simulink model "r2_b16a4x512f"  (R2012b)
settings: Solver=VariableStepDiscrete  SolverMode=SingleTasking  StartTime=0.0  StopTime=1  RelTol=1e-3
undefined symbols (not defined in the file): fft_stages, n_bits_ants, n_bits_xengs
libraries: xbsIndex_r4 x27410, casper_library_misc x230, xbsReplacements_r4 x24, casper_library_delays x8, xps_library x5, casper_library_communications x4
(part 69 of 229)

== system r2_b16a4x512f/sys0/vacc/bus_relational ==
  a : Inport
  b : Inport  Port=2
  a_debus : Subsystem  AncestorBlock=casper_library_flow_control/bus_expand  mask(bus_expand){mode=divisions of arbitrary size, outputNum=1, outputWidth=[1  1  1  1  1  1  1  1  1  1  1  1  1  1  1  1  1  1  1], outputBinaryPt=[0  0  0  0  0  0  0  0  0  0  0  0  0  0  0  0  0  0  0], outputArithmeticType=[0  0  0  0  0  0  0  0  0  0  0  0  0  0  0  0  0  0  0], show_format=on, outputToWorkspace=off, variablePrefix=, outputToModelAsWell=on}
      mask prompts: outputNum "Number of outputs:"; outputWidth "Output width [msb ... lsb]:"; outputBinaryPt "Output binary point position [msb ... lsb]:"; outputArithmeticType "Output arithmetic type (ufix=0, fix=1, bool=2) [msb ... lsb]:"; show_format "Print format string?"; outputToWorkspace "Output to workspace?"; variablePrefix "Variable name prefix:"; outputToModelAsWell "Output to model as well?"
      mask help:
      | Expands a 'bus' made using a bus_create or Xilinx
      | concat block.
      | The input will be divided into the specified number
      | of outputs with the specified arithmetic types.
      | Divisions are made from most significant bit.
      mask init: same as r2_b16a4x512f/bus_expand
      settings: AttributesFormatString=19 outputs: uf1.0,uf1.0,uf1.0,uf1.0,uf1.0,uf1.0,uf1.0,uf1.0,uf1.0,uf1.0,uf1.0,uf1.0,uf1.0,uf1.0,uf1.0,uf1.0,uf1.0,uf1.0,uf1.0,
      mask TypeOptions mode: divisions of equal size | divisions of arbitrary size
      mask Callback mode: bus_expand_callback();
      mask Callback outputWidth: bus_expand_callback();
      mask Callback outputToWorkspace: bus_expand_callback();
  b_debus : Subsystem  AncestorBlock=casper_library_flow_control/bus_expand  mask(bus_expand){mode=divisions of arbitrary size, outputNum=1, outputWidth=[1  1  1  1  1  1  1  1  1  1  1  1  1  1  1  1  1  1  1], outputBinaryPt=[0  0  0  0  0  0  0  0  0  0  0  0  0  0  0  0  0  0  0], outputArithmeticType=[0  0  0  0  0  0  0  0  0  0  0  0  0  0  0  0  0  0  0], show_format=on, outputToWorkspace=off, variablePrefix=, outputToModelAsWell=on}
      mask prompts: outputNum "Number of outputs:"; outputWidth "Output width [msb ... lsb]:"; outputBinaryPt "Output binary point position [msb ... lsb]:"; outputArithmeticType "Output arithmetic type (ufix=0, fix=1, bool=2) [msb ... lsb]:"; show_format "Print format string?"; outputToWorkspace "Output to workspace?"; variablePrefix "Variable name prefix:"; outputToModelAsWell "Output to model as well?"
      mask help:
      | Expands a 'bus' made using a bus_create or Xilinx
      | concat block.
      | The input will be divided into the specified number
      | of outputs with the specified arithmetic types.
      | Divisions are made from most significant bit.
      mask init: same as r2_b16a4x512f/bus_expand
      settings: AttributesFormatString=19 outputs: uf1.0,uf1.0,uf1.0,uf1.0,uf1.0,uf1.0,uf1.0,uf1.0,uf1.0,uf1.0,uf1.0,uf1.0,uf1.0,uf1.0,uf1.0,uf1.0,uf1.0,uf1.0,uf1.0,
      mask TypeOptions mode: divisions of equal size | divisions of arbitrary size
      mask Callback mode: bus_expand_callback();
      mask Callback outputWidth: bus_expand_callback();
      mask Callback outputToWorkspace: bus_expand_callback();
  bussify : Subsystem  AncestorBlock=casper_library_flow_control/bus_create  mask(bus_create){inputNum=19}
      mask prompts: inputNum "Number of inputs:"
      mask init:
      | bus_create_init(gcb,...
      |     'inputNum', inputNum);
  relational{1..19} (19 alike) : xbsIndex_r4/Relational  mode=a!=b  en=off  latency=0  dbl_ovrd=off  block_type=relational
  a!=b : Outport
  wires:
  a/1 -> a_debus/1(bus_in)
  b/1 -> b_debus/1(bus_in)
  a_debus/1(msb_out19) -> relational1/1
  b_debus/1(msb_out19) -> relational1/2
  a_debus/2(out18) -> relational2/1
  b_debus/2(out18) -> relational2/2
  a_debus/3(out17) -> relational3/1
  b_debus/3(out17) -> relational3/2
  a_debus/4(out16) -> relational4/1
  b_debus/4(out16) -> relational4/2
  a_debus/5(out15) -> relational5/1
  b_debus/5(out15) -> relational5/2
  a_debus/6(out14) -> relational6/1
  b_debus/6(out14) -> relational6/2
  a_debus/7(out13) -> relational7/1
  b_debus/7(out13) -> relational7/2
  a_debus/8(out12) -> relational8/1
  b_debus/8(out12) -> relational8/2
  a_debus/9(out11) -> relational9/1
  b_debus/9(out11) -> relational9/2
  a_debus/10(out10) -> relational10/1
  b_debus/10(out10) -> relational10/2
  a_debus/11(out9) -> relational11/1
  b_debus/11(out9) -> relational11/2
  a_debus/12(out8) -> relational12/1
  b_debus/12(out8) -> relational12/2
  a_debus/13(out7) -> relational13/1
  b_debus/13(out7) -> relational13/2
  a_debus/14(out6) -> relational14/1
  b_debus/14(out6) -> relational14/2
  a_debus/15(out5) -> relational15/1
  b_debus/15(out5) -> relational15/2
  a_debus/16(out4) -> relational16/1
  b_debus/16(out4) -> relational16/2
  a_debus/17(out3) -> relational17/1
  b_debus/17(out3) -> relational17/2
  a_debus/18(out2) -> relational18/1
  b_debus/18(out2) -> relational18/2
  a_debus/19(lsb_out1) -> relational19/1
  b_debus/19(lsb_out1) -> relational19/2
  relational1/1 -> bussify/1(in1)
  relational2/1 -> bussify/2(in2)
  relational3/1 -> bussify/3(in3)
  relational4/1 -> bussify/4(in4)
  relational5/1 -> bussify/5(in5)
  relational6/1 -> bussify/6(in6)
  relational7/1 -> bussify/7(in7)
  relational8/1 -> bussify/8(in8)
  relational9/1 -> bussify/9(in9)
  relational10/1 -> bussify/10(in10)
  relational11/1 -> bussify/11(in11)
  relational12/1 -> bussify/12(in12)
  relational13/1 -> bussify/13(in13)
  relational14/1 -> bussify/14(in14)
  relational15/1 -> bussify/15(in15)
  relational16/1 -> bussify/16(in16)
  relational17/1 -> bussify/17(in17)
  relational18/1 -> bussify/18(in18)
  relational19/1 -> bussify/19(in19)
  bussify/1(bus_out) -> a!=b/1

== system r2_b16a4x512f/sys0/vacc/flag_sampler ==
  sync : Inport
  in : Inport  Port=2
  enable : Inport  Port=3
  Constant3 : xbsIndex_r4/Constant  const=period-1  gui_display_data_type=Fixed-point  arith_type=Unsigned  n_bits=ceil(log2(period))  bin_pt=0  preci_type=Single  exp_width=8  frac_width=24  explicit_period=on  period=1  equ=P=C  opselect=C  inp2=PCIN>>17  opr=+  inp1=P  carry=CIN  dbl_ovrd=off  block_type=constant
  Counter4 : xbsIndex_r4/Counter  cnt_type=Free Running  cnt_to=Inf  operation=Up  start_count=0  cnt_by_val=1  arith_type=Unsigned  n_bits=ceil(log2(period))  bin_pt=0  load_pin=off  rst=on  en=on  explicit_period=on  period=1  dbl_ovrd=off  use_behavioral_HDL=off  implementation=Fabric  use_rpm=on  block_type=counter
      settings: xl_area=[0, 0, 0, 0, 0, 0, 0]
  Delay10 : xbsIndex_r4/Delay  rst=off  infoeditControl=Selection of Reset will increase slice count due to use of real FFs and instead of SRLs  en=off  latency=1  dbl_ovrd=off  reg_retiming=on  block_type=delay
      settings: xl_area=[0, 0, 0, 0, 0, 0, 0]
  Logical : xbsIndex_r4/Logical  logical_function=OR  inputs=2  en=off  latency=0  precision=Full  arith_type=Unsigned  n_bits=16  bin_pt=0  align_bp=on  dbl_ovrd=off  block_type=logical
  Register : xbsIndex_r4/Register  init=0  rst=off  en=on  dbl_ovrd=off  block_type=register
  Relational : xbsIndex_r4/Relational  mode=a>=b  en=off  latency=0  dbl_ovrd=off  block_type=relational
      settings: xl_area=[0, 0, 0, 0, 0, 0, 0]  block_version=10.1.3
  out : Outport
  sample_out : Outport  Port=2
  wires:
  enable/1 -> Counter4/2
  Relational/1 -> Logical/1
  Constant3/1 -> Relational/2
  Counter4/1 -> Relational/1
  Logical/1 -> Delay10/1, Counter4/1
  sync/1 -> Logical/2
  Register/1 -> out/1
  in/1 -> Register/1
  Delay10/1 -> sample_out/1, Register/2

== system r2_b16a4x512f/sys0/vacc/mcnt_sampler ==
  sync : Inport
  in : Inport  Port=2
  enable : Inport  Port=3
  Constant3 : xbsIndex_r4/Constant  const=period-1  gui_display_data_type=Fixed-point  arith_type=Unsigned  n_bits=ceil(log2(period))  bin_pt=0  preci_type=Single  exp_width=8  frac_width=24  explicit_period=on  period=1  equ=P=C  opselect=C  inp2=PCIN>>17  opr=+  inp1=P  carry=CIN  dbl_ovrd=off  block_type=constant
  Counter4 : xbsIndex_r4/Counter  cnt_type=Free Running  cnt_to=Inf  operation=Up  start_count=0  cnt_by_val=1  arith_type=Unsigned  n_bits=ceil(log2(period))  bin_pt=0  load_pin=off  rst=on  en=on  explicit_period=on  period=1  dbl_ovrd=off  use_behavioral_HDL=off  implementation=Fabric  use_rpm=on  block_type=counter
      settings: xl_area=[0, 0, 0, 0, 0, 0, 0]
  Delay10 : xbsIndex_r4/Delay  rst=off  infoeditControl=Selection of Reset will increase slice count due to use of real FFs and instead of SRLs  en=off  latency=1  dbl_ovrd=off  reg_retiming=on  block_type=delay
      settings: xl_area=[0, 0, 0, 0, 0, 0, 0]
  Logical : xbsIndex_r4/Logical  logical_function=OR  inputs=2  en=off  latency=0  precision=Full  arith_type=Unsigned  n_bits=16  bin_pt=0  align_bp=on  dbl_ovrd=off  block_type=logical
  Register : xbsIndex_r4/Register  init=0  rst=off  en=on  dbl_ovrd=off  block_type=register
  Relational : xbsIndex_r4/Relational  mode=a>=b  en=off  latency=0  dbl_ovrd=off  block_type=relational
      settings: xl_area=[0, 0, 0, 0, 0, 0, 0]  block_version=10.1.3
  out : Outport
  sample_out : Outport  Port=2
  wires:
  enable/1 -> Counter4/2
  Relational/1 -> Logical/1
  Constant3/1 -> Relational/2
  Counter4/1 -> Relational/1
  Logical/1 -> Delay10/1, Counter4/1
  sync/1 -> Logical/2
  Register/1 -> out/1
  in/1 -> Register/1
  Delay10/1 -> sample_out/1, Register/2

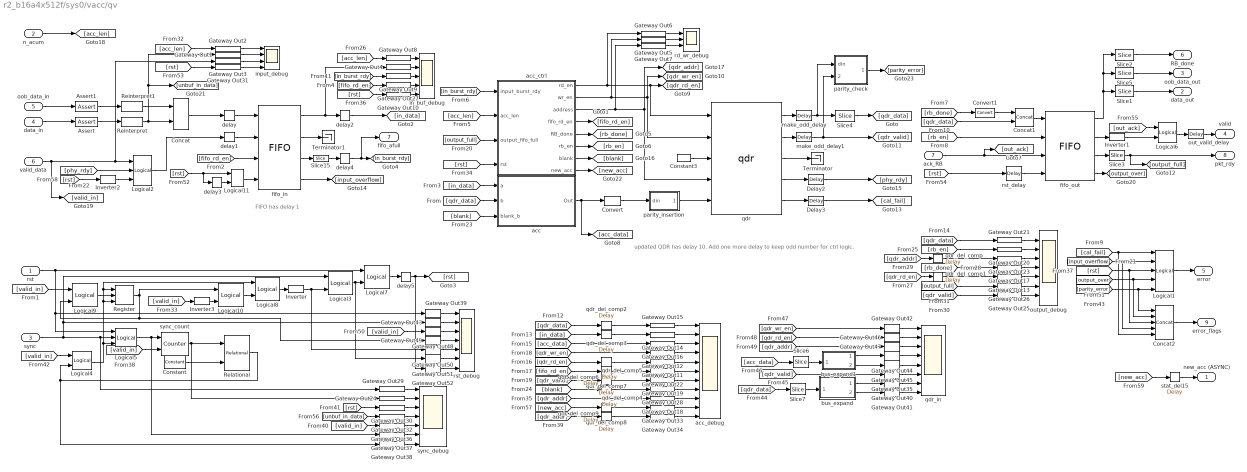
== system r2_b16a4x512f/sys0/vacc/qv ==
  note: FIFO has delay 1
  note: updated QDR has delay 10.
      | Add one more delay to keep
      | odd number for ctrl logic.
  rst : Inport
  n_acum : Inport  Port=2
  sync : Inport  Port=3
  data_in : Inport  Port=4
  oob_data_in : Inport  Port=5
  valid_data : Inport  Port=6
  ack_RB : Inport  Port=7
  Assert : xbsIndex_r4/Assert  assert_type=on  type_source=Explicitly  gui_display_data_type=Fixed-point  arith_type=Unsigned  n_bits=n_bits*2^n_inputs  bin_pt=0  preci_type=Single  exp_width=8  frac_width=24  assert_rate=off  rate_source=Explicitly  period=1  output_port=on  block_type=assert
      settings: block_version=10.1.3
  Assert1 : xbsIndex_r4/Assert  assert_type=on  type_source=Explicitly  gui_display_data_type=Fixed-point  arith_type=Unsigned  n_bits=4  bin_pt=0  preci_type=Single  exp_width=8  frac_width=24  assert_rate=on  rate_source=Explicitly  period=1  output_port=on  block_type=assert
      settings: infoedit=Asserts a user-defined sample rate and/or type on a signal.<P><P>Hardware notes: In hardware this block costs nothing.  block_version=10.1.3
  Concat : xbsIndex_r4/Concat  num_inputs=2  dbl_ovrd=off  block_type=concat
      settings: block_version=9.2.01
  Concat1 : xbsIndex_r4/Concat  num_inputs=2  dbl_ovrd=off  block_type=concat
      settings: block_version=9.2.01
  Concat2 : xbsIndex_r4/Concat  num_inputs=5  dbl_ovrd=off  block_type=concat
  Constant : xbsIndex_r4/Constant  const=vector_len-1  gui_display_data_type=Fixed-point  arith_type=Unsigned  n_bits=vector_bits  bin_pt=0  preci_type=Single  exp_width=8  frac_width=24  explicit_period=on  period=1  equ=P=C  opselect=C  inp2=PCIN>>17  opr=+  inp1=P  carry=CIN  dbl_ovrd=off  block_type=constant
  Constant3 : xbsIndex_r4/Constant  const=(2^4)-1  gui_display_data_type=Fixed-point  arith_type=Unsigned  n_bits=4  bin_pt=0  preci_type=Single  exp_width=8  frac_width=24  explicit_period=on  period=1  equ=P=C  opselect=C  inp2=PCIN>>17  opr=+  inp1=P  carry=CIN  dbl_ovrd=off  block_type=constant
      settings: block_version=9.2.01
  Convert : xbsIndex_r4/Convert  gui_display_data_type=Fixed-point  arith_type=Unsigned  n_bits=71  bin_pt=0  float_type=Single  exp_bits=8  fraction_bits=24  quantization=Truncate  overflow=Wrap  en=off  latency=0  dbl_ovrd=off  pipeline=off  block_type=convert
  Convert1 : xbsIndex_r4/Convert  gui_display_data_type=Fixed-point  arith_type=Unsigned  n_bits=1  bin_pt=0  float_type=Single  exp_bits=8  fraction_bits=24  quantization=Truncate  overflow=Wrap  en=off  latency=0  dbl_ovrd=off  pipeline=off  block_type=convert
      settings: xl_area=[0, 0, 0, 0, 0, 0, 0]  block_version=9.2.01
  Delay2 : xbsIndex_r4/Delay  rst=off  infoeditControl=Selection of Reset will increase slice count due to use of real FFs and instead of SRLs  en=off  latency=1  dbl_ovrd=off  reg_retiming=on  block_type=delay
  Delay3 : xbsIndex_r4/Delay  rst=off  infoeditControl=Selection of Reset will increase slice count due to use of real FFs and instead of SRLs  en=off  latency=1  dbl_ovrd=off  reg_retiming=on  block_type=delay
  Gateway Out{1..52} (52 alike) : xbsIndex_r4/Gateway Out  inherit_from_input=off  hdl_port=off  timing_constraint=None  locs_specified=off  LOCs={}  UseAsDAC=off  DACChannel='1'  block_type=gatewayout
      settings: infoedit="Gateway out block.  Converts Xilinx fixed point inputs into ouputs of type Simulink integer, double, or fixed point.<P><P>Hardware notes:  In hardware these blocks become top level output ports or are discarded, depending on how they are configured."  xl_area=[0, 0, 0, 0, 0, 0, 0]  block_version=10.1.3
  Inverter{,1..3} (4 alike) : xbsIndex_r4/Inverter  en=off  latency=0  dbl_ovrd=off  block_type=inv
  Logical1 : xbsIndex_r4/Logical  logical_function=OR  inputs=5  en=off  latency=1  precision=Full  arith_type=Unsigned  n_bits=16  bin_pt=0  align_bp=on  dbl_ovrd=off  block_type=logical
  Logical{3..4,6,9..10} (5 alike) : xbsIndex_r4/Logical  logical_function=AND  inputs=2  en=off  latency=0  precision=Full  arith_type=Unsigned  n_bits=16  bin_pt=0  align_bp=on  dbl_ovrd=off  block_type=logical
  Logical11 : xbsIndex_r4/Logical  logical_function=OR  inputs=2  en=off  latency=0  precision=Full  arith_type=Unsigned  n_bits=16  bin_pt=0  align_bp=on  dbl_ovrd=off  block_type=logical
  Logical2 : xbsIndex_r4/Logical  logical_function=AND  inputs=3  en=off  latency=0  precision=Full  arith_type=Unsigned  n_bits=16  bin_pt=0  align_bp=on  dbl_ovrd=off  block_type=logical
  Logical5 : xbsIndex_r4/Logical  logical_function=OR  inputs=3  en=off  latency=0  precision=Full  arith_type=Unsigned  n_bits=16  bin_pt=0  align_bp=on  dbl_ovrd=off  block_type=logical
  Logical7 : xbsIndex_r4/Logical  logical_function=OR  inputs=2  en=off  latency=0  precision=Full  arith_type=Unsigned  n_bits=16  bin_pt=0  align_bp=on  dbl_ovrd=off  block_type=logical
  Logical8 : xbsIndex_r4/Logical  logical_function=OR  inputs=2  en=off  latency=0  precision=Full  arith_type=Unsigned  n_bits=16  bin_pt=0  align_bp=on  dbl_ovrd=off  block_type=logical
  Register : xbsIndex_r4/Register  init=0  rst=on  en=on  dbl_ovrd=off  block_type=register
      settings: block_version=11.4
  Reinterpret : xbsIndex_r4/Reinterpret  force_arith_type=on  arith_type=Unsigned  force_bin_pt=on  bin_pt=0  block_type=reinterpret
      settings: block_version=9.2.01
  Reinterpret1 : xbsIndex_r4/Reinterpret  force_arith_type=on  arith_type=Unsigned  force_bin_pt=on  bin_pt=0  block_type=reinterpret
      settings: infoedit="Changes signal type without altering the binary representation.   You can changed the signal between signed and unsigned, and relocate the binary point.<P><P>Hardware notes: In hardware this block costs nothing.<P><P>Example:  Suppose the input is 6 bits wide, signed, with 2 fractional bits, and the output is forced to unsigned with 0 fractional bits.  Then an input of -2.0 (1110.00 in binary 2's complement) becomes an output of 56 (111000 in binary)."  block_version=9.2.01
  Relational : xbsIndex_r4/Relational  mode=a>=b  en=off  latency=0  dbl_ovrd=off  block_type=relational
      settings: block_version=10.1.3
  Slice1 : xbsIndex_r4/Slice  nbits=n_bits*2^n_inputs  boolean_output=off  mode=Lower Bit Location + Width  bit1=96  base1=MSB of Input  bit0=0  base0=LSB of Input  dbl_ovrd=off  block_type=slice
      settings: block_version=9.2.01
  Slice15 : xbsIndex_r4/Slice  nbits=1  boolean_output=on  mode=Upper Bit Location + Width  bit1=0  base1=MSB of Input  bit0=0  base0=LSB of Input  dbl_ovrd=off  block_type=slice
      settings: infoedit="Extracts a given range of bits from each input sample and presents it at the output.  The output type is ordinarily unsigned with binary point at zero, but can be Boolean when the slice is one bit wide.<P><P>Hardware notes: In hardware this block costs nothing."  block_version=9.2.01
  Slice2 : xbsIndex_r4/Slice  nbits=1  boolean_output=on  mode=Lower Bit Location + Width  bit1=-1  base1=MSB of Input  bit0=(2^n_inputs*n_bits)+4  base0=LSB of Input  dbl_ovrd=off  block_type=slice
      settings: block_version=9.2.01
  Slice3 : xbsIndex_r4/Slice  nbits=1  boolean_output=on  mode=Upper Bit Location + Width  bit1=0  base1=MSB of Input  bit0=0  base0=LSB of Input  dbl_ovrd=off  block_type=slice
      settings: infoedit="Extracts a given range of bits from each input sample and presents it at the output.  The output type is ordinarily unsigned with binary point at zero, but can be Boolean when the slice is one bit wide.<P><P>Hardware notes: In hardware this block costs nothing."  block_version=9.2.01
  Slice4 : xbsIndex_r4/Slice  nbits=(n_bits*2^n_inputs)+4  boolean_output=off  mode=Lower Bit Location + Width  bit1=96  base1=MSB of Input  bit0=0  base0=LSB of Input  dbl_ovrd=off  block_type=slice
      settings: block_version=9.2.01
  Slice5 : xbsIndex_r4/Slice  nbits=4  boolean_output=off  mode=Lower Bit Location + Width  bit1=96  base1=MSB of Input  bit0=n_bits*n_inputs  base0=LSB of Input  dbl_ovrd=off  block_type=slice
      settings: block_version=9.2.01
  Slice6 : xbsIndex_r4/Slice  nbits=(n_bits*2^n_inputs)  boolean_output=off  mode=Lower Bit Location + Width  bit1=96  base1=MSB of Input  bit0=0  base0=LSB of Input  dbl_ovrd=off  block_type=slice
      settings: block_version=9.2.01
  Slice7 : xbsIndex_r4/Slice  nbits=(n_bits*2^n_inputs)  boolean_output=off  mode=Lower Bit Location + Width  bit1=96  base1=MSB of Input  bit0=0  base0=LSB of Input  dbl_ovrd=off  block_type=slice
      settings: block_version=9.2.01
  Terminator : Terminator
  Terminator1 : Terminator
  acc : Subsystem  mask{n_inputs=2^n_inputs, n_bits=n_bits}
      mask prompts: n_inputs "Simultaneous inputs"; n_bits "Data width"
  acc_ctrl : Subsystem  mask{delay_qdr=11, delay_in_fifo=1, delay_adder=2}
      mask prompts: delay_qdr "delay qdr"
      mask help: QDR delay must be odd (9 is ok, 11 is ok, 10 is not).
  acc_debug : Scope  NumInputPorts=11
      settings: TimeRange=57000  YMin=0~0~0~0~0~0~0~1~1540~-1~1540  YMax=7.5e+15~7.5e+15~7.5e+15~1~1~1~1~1~1555~1~1555  SaveName=ScopeData4
  bus_expand : Subsystem  AncestorBlock=casper_library_flow_control/bus_expand  mask(bus_expand){mode=divisions of arbitrary size, outputNum=1, outputWidth=[32 32], outputBinaryPt=[14 14], outputArithmeticType=[1 1], show_format=off, outputToWorkspace=off, variablePrefix=out, outputToModelAsWell=on}
      mask prompts: outputNum "Number of outputs:"; outputWidth "Output width [msb ... lsb]:"; outputBinaryPt "Output binary point position [msb ... lsb]:"; outputArithmeticType "Output arithmetic type (ufix=0, fix=1, bool=2) [msb ... lsb]:"; show_format "Print format string?"; outputToWorkspace "Output to workspace?"; variablePrefix "Variable name prefix:"; outputToModelAsWell "Output to model as well?"
      mask help:
      | Expands a 'bus' made using a bus_create or Xilinx
      | concat block.
      | The input will be divided into the specified number
      | of outputs with the specified arithmetic types.
      | Divisions are made from most significant bit.
      mask init: same as r2_b16a4x512f/bus_expand
      settings: AttributesFormatString=2 outputs
      mask TypeOptions mode: divisions of equal size | divisions of arbitrary size
      mask Callback mode: bus_expand_callback();
      mask Callback outputWidth: bus_expand_callback();
      mask Callback outputToWorkspace: bus_expand_callback();
  bus_expand1 : Subsystem  AncestorBlock=casper_library_flow_control/bus_expand  mask(bus_expand){mode=divisions of arbitrary size, outputNum=1, outputWidth=[32 32], outputBinaryPt=[14 14], outputArithmeticType=[1 1], show_format=off, outputToWorkspace=off, variablePrefix=out, outputToModelAsWell=on}
      mask prompts: outputNum "Number of outputs:"; outputWidth "Output width [msb ... lsb]:"; outputBinaryPt "Output binary point position [msb ... lsb]:"; outputArithmeticType "Output arithmetic type (ufix=0, fix=1, bool=2) [msb ... lsb]:"; show_format "Print format string?"; outputToWorkspace "Output to workspace?"; variablePrefix "Variable name prefix:"; outputToModelAsWell "Output to model as well?"
      mask help:
      | Expands a 'bus' made using a bus_create or Xilinx
      | concat block.
      | The input will be divided into the specified number
      | of outputs with the specified arithmetic types.
      | Divisions are made from most significant bit.
      mask init: same as r2_b16a4x512f/bus_expand
      settings: AttributesFormatString=2 outputs
      mask TypeOptions mode: divisions of equal size | divisions of arbitrary size
      mask Callback mode: bus_expand_callback();
      mask Callback outputWidth: bus_expand_callback();
      mask Callback outputToWorkspace: bus_expand_callback();
  delay{,1..5} (6 alike) : xbsIndex_r4/Delay  rst=off  infoeditControl=Selection of Reset will increase slice count due to use of real FFs and instead of SRLs  en=off  latency=1  dbl_ovrd=off  reg_retiming=on  block_type=delay
  fifo_in : xbsIndex_r4/FIFO  mem_type=Distributed RAM  performance_options=Standard_FIFO  infoedit1=Available only for V4, V5, V6, V7, K7, A7 and Zynq devices.  embedded_registers=off  depth=64  percent_nbits=1  rst=on  en=off  use_dcount=off  use_percent_full_port=on  use_almost_empty=off  almost_empty_thresh=2  use_almost_full=off  almost_full_thresh=14  dbl_ovrd=off  explicit_period=off  block_type=fifo
      settings: block_version=10.1.3
  fifo_out : xbsIndex_r4/FIFO  mem_type=Block RAM  performance_options=Standard_FIFO  infoedit1=Available only for V4, V5, V6, V7, K7, A7 and Zynq devices.  embedded_registers=off  depth=1K  percent_nbits=1  rst=on  en=off  use_dcount=off  use_percent_full_port=on  use_almost_empty=off  almost_empty_thresh=2  use_almost_full=off  almost_full_thresh=14  dbl_ovrd=off  explicit_period=off  block_type=fifo
      settings: block_version=10.1.3
  in_buf_debug : Scope  NumInputPorts=5
      settings: YMin=7.6~-1~-1~-1~-1  YMax=8.4~1~1~1~1  SaveName=ScopeData2
  input_debug : Scope  NumInputPorts=4
      settings: YMin=12000~0~-5~-5  YMax=13300~1~5~5
  make_odd_delay : xbsIndex_r4/Delay  rst=off  infoeditControl=Selection of Reset will increase slice count due to use of real FFs and instead of SRLs  en=off  latency=1  dbl_ovrd=off  reg_retiming=on  block_type=delay
  make_odd_delay1 : xbsIndex_r4/Delay  rst=off  infoeditControl=Selection of Reset will increase slice count due to use of real FFs and instead of SRLs  en=off  latency=1  dbl_ovrd=off  reg_retiming=on  block_type=delay
  out_valid_delay : xbsIndex_r4/Delay  rst=off  infoeditControl=Selection of Reset will increase slice count due to use of real FFs and instead of SRLs  en=off  latency=1  dbl_ovrd=off  reg_retiming=on  block_type=delay
  output_debug : Scope  NumInputPorts=7
      settings: YMin=0~0~0~-1~0~-1~0.95  YMax=2.5e+16~1~9000~1~1~1~1.05  SaveName=ScopeData3
  parity_check : Subsystem
  parity_insertion : Subsystem
  qdr : xps_library/qdr  Tag=xps:qdr  which_qdr=qdr0  qdr_awidth=vector_bits  use_sniffer=on
      link override convert_be: n_bits=8
      link override convert_data_in: n_bits=72
      link override convert_data_in1: n_bits=72
      link override extract_parity: bitexpr=b = {a[71:0]}  arith_type1=Unsigned  arith_type2=Unsigned  arith_type3=Unsigned  arith_type4=Unsigned
      link override insert_parity: bitexpr=b = {a[71:0]}  arith_type1=Unsigned  arith_type2=Unsigned  arith_type3=Unsigned  arith_type4=Unsigned
      link override qdr_sim_model/Dual Port RAM: depth=2^qdr_awidth  initVector=[1:2^qdr_awidth]  distributed_mem=Block RAM  init_a=0  init_b=0  rst_a=off  rst_b=off  en_a=off  en_b=off  latency=1  write_mode_A=Read Before Write  write_mode_B=Read Before Write  dbl_ovrd=off  optimize=Area
      link override qdr_sim_model/sim_data_in: n_bits=72
      link override r2_2f_4x_4a_4k_r366_vacc0_qv_qdr_data_out: n_bits=72
      link override r2_4a4x128f_sys0_vacc_qv_qdr_data_out: n_bits=72
      link override r2_4a4x2kf_sys0_vacc_qv_qdr_data_out: n_bits=72
      link override r2_b4a4x256f_4gbe_sys0_vacc_qv_qdr_data_out: n_bits=72
      link override r2_b4a4x256f_sys0_vacc_qv_qdr_data_out: n_bits=72
      link override x_nd_full_sys0_vacc0_qv_qdr_data_out: n_bits=72
      link override x_nd_full_sys2_vacc0_qv_qdr_data_out: n_bits=72
      link override x_nd_inc_sys2_vacc0_qv_qdr_data_out: n_bits=72
      link override x_new_bc_sys0_vacc0_qv_qdr_data_out: n_bits=72
      link override xeng_sim_vacc0_qv_qdr_data_out: n_bits=72
  qdr_del_comp : xbsIndex_r4/Delay  rst=off  infoeditControl=Selection of Reset will increase slice count due to use of real FFs and instead of SRLs  en=off  latency=11  dbl_ovrd=off  reg_retiming=on  block_type=delay
  qdr_del_comp1 : xbsIndex_r4/Delay  rst=off  infoeditControl=Selection of Reset will increase slice count due to use of real FFs and instead of SRLs  en=off  latency=11  dbl_ovrd=off  reg_retiming=on  block_type=delay
  qdr_del_comp{2..4,6} (4 alike) : xbsIndex_r4/Delay  rst=off  infoeditControl=Selection of Reset will increase slice count due to use of real FFs and instead of SRLs  en=off  latency=2  dbl_ovrd=off  reg_retiming=on  block_type=delay
  qdr_del_comp5 : xbsIndex_r4/Delay  rst=off  infoeditControl=Selection of Reset will increase slice count due to use of real FFs and instead of SRLs  en=off  latency=13  dbl_ovrd=off  reg_retiming=on  block_type=delay
  qdr_del_comp7 : xbsIndex_r4/Delay  rst=off  infoeditControl=Selection of Reset will increase slice count due to use of real FFs and instead of SRLs  en=off  latency=3  dbl_ovrd=off  reg_retiming=on  block_type=delay
  qdr_del_comp8 : xbsIndex_r4/Delay  rst=off  infoeditControl=Selection of Reset will increase slice count due to use of real FFs and instead of SRLs  en=off  latency=13  dbl_ovrd=off  reg_retiming=on  block_type=delay
  qdr_del_comp9 : xbsIndex_r4/Delay  rst=off  infoeditControl=Selection of Reset will increase slice count due to use of real FFs and instead of SRLs  en=off  latency=13  dbl_ovrd=off  reg_retiming=on  block_type=delay
  qdr_in : Scope  NumInputPorts=8
      settings: TimeRange=57000  YMin=0~0~2407.5~0~-1~0~0~0  YMax=1~1~2422.5~100~1~1~200~0.0075  SaveName=ScopeData14
  rd_wr_debug : Scope  NumInputPorts=3
      settings: YMin=0~0~0  YMax=1~1~1050
  rst_debug : Scope  NumInputPorts=7
      settings: YMin=7.6~-1~-1~-1~-1~-5~-5  YMax=8.4~1~1~1~1~5~5  SaveName=ScopeData16
  rst_delay : xbsIndex_r4/Delay  rst=off  infoeditControl=Selection of Reset will increase slice count due to use of real FFs and instead of SRLs  en=off  latency=1  dbl_ovrd=off  reg_retiming=on  block_type=delay
  stat_del15 : xbsIndex_r4/Delay  rst=off  infoeditControl=Selection of Reset will increase slice count due to use of real FFs and instead of SRLs  en=off  latency=1  dbl_ovrd=off  reg_retiming=on  block_type=delay
  sync_count : xbsIndex_r4/Counter  cnt_type=Free Running  cnt_to=Inf  operation=Up  start_count=0  cnt_by_val=1  arith_type=Unsigned  n_bits=vector_bits  bin_pt=0  load_pin=off  rst=on  en=on  explicit_period=on  period=1  dbl_ovrd=off  use_behavioral_HDL=on  implementation=Fabric  use_rpm=on  block_type=counter
  sync_debug : Scope  NumInputPorts=7
      settings: YMin=-1~1090~-1~-1~0~-1~-1  YMax=1~1090~1~1~1~1~1  SaveName=ScopeData7
  new_acc (ASYNC) : Outport
  data_out : Outport  Port=2
  oob_data_out : Outport  Port=3
  valid : Outport  Port=4
  error : Outport  Port=5
  RB_done : Outport  Port=6
  fifo_afull : Outport  Port=7
  pkt_rdy : Outport  Port=8
  error_flags : Outport  Port=9
  wires:
  delay5/1 -> Gateway Out52/1, [rst]
  delay4/1 -> [in_burst_rdy], fifo_afull/1
  delay2/1 -> [in_data]
  qdr_del_comp9/1 -> Gateway Out34/1
  Gateway Out34/1 -> acc_debug/11
  [qdr_addr] -> qdr_del_comp9/1
  qdr_del_comp1/1 -> Gateway Out13/1
  qdr_del_comp/1 -> Gateway Out23/1
  make_odd_delay1/1 -> [qdr_valid], parity_check/2(valid)
  make_odd_delay/1 -> parity_check/1(din), Slice4/1
  Reinterpret1/1 -> Concat/1
  Reinterpret/1 -> Gateway Out1/1, [unbuf_in_data], Concat/2
  Assert1/1 -> Reinterpret1/1
  Assert/1 -> Reinterpret/1
  [in_data] -> acc/1(a)
  [rst] -> Gateway Out10/1
  Gateway Out10/1 -> in_buf_debug/5
  Gateway Out18/1 -> acc_debug/9
  [qdr_addr] -> Gateway Out18/1
  [rst] -> acc_ctrl/4(rst)
  [acc_len] -> Gateway Out2/1
  [acc_len] -> Gateway Out8/1
  [acc_len] -> acc_ctrl/2(acc_len)
  oob_data_in/1 -> Assert1/1
  n_acum/1 -> [acc_len]
  Gateway Out23/1 -> output_debug/3
  [qdr_addr] -> qdr_del_comp/1
  Gateway Out26/1 -> output_debug/6
  [rb_done] -> Gateway Out17/1
  [rb_en] -> Gateway Out20/1
  Gateway Out25/1 -> output_debug/7
  Gateway Out13/1 -> output_debug/5
  Gateway Out17/1 -> output_debug/4
  Gateway Out20/1 -> output_debug/2
  Gateway Out21/1 -> output_debug/1
  [output_full] -> Gateway Out26/1
  [qdr_valid] -> Gateway Out25/1
  [qdr_rd_en] -> qdr_del_comp1/1
  [qdr_data] -> Gateway Out21/1
  Gateway Out28/1 -> acc_debug/8
  Gateway Out19/1 -> acc_debug/7
  Gateway Out22/1 -> acc_debug/6
  Gateway Out11/1 -> acc_debug/5
  Gateway Out12/1 -> acc_debug/4
  Gateway Out16/1 -> acc_debug/3
  Gateway Out14/1 -> acc_debug/2
  Gateway Out15/1 -> acc_debug/1
  [blank] -> qdr_del_comp4/1
  [blank] -> acc/3(blank_b)
  acc_ctrl/7(blank) -> [blank]
  [qdr_data] -> acc/2(b)
  fifo_out/4 -> [output_over]
  qdr/3 -> Terminator/1
  [phy_rdy] -> Logical2/2
  Logical2/1 -> delay1/1
  Delay3/1 -> [cal_fail]
  Delay2/1 -> [phy_rdy]
  qdr/4 -> Delay2/1
  fifo_in/4 -> [input_overflow]
  qdr/5 -> Delay3/1
  Logical1/1 -> error/1
  acc_ctrl/5(RB_done) -> [rb_done]
  acc_ctrl/6(rb_en) -> [rb_en]
  fifo_out/3 -> Slice3/1
  [output_full] -> acc_ctrl/3(output_fifo_full)
  [qdr_valid] -> qdr_del_comp6/1
  qdr/2 -> make_odd_delay1/1
  [qdr_wr_en] -> Gateway Out12/1
  [fifo_rd_en] -> qdr_del_comp7/1
  [qdr_rd_en] -> qdr_del_comp5/1
  [acc_data] -> Gateway Out16/1
  [in_data] -> qdr_del_comp3/1
  [qdr_data] -> qdr_del_comp2/1
  Slice5/1 -> oob_data_out/1
  [in_burst_rdy] -> Gateway Out9/1
  [fifo_rd_en] -> Gateway Out27/1
  Gateway Out27/1 -> in_buf_debug/4
  Gateway Out9/1 -> in_buf_debug/3
  Gateway Out4/1 -> in_buf_debug/2
  Gateway Out8/1 -> in_buf_debug/1
  Gateway Out3/1 -> input_debug/3
  Gateway Out1/1 -> input_debug/2
  Gateway Out2/1 -> input_debug/1
  acc/1(Out) -> Convert/1, [acc_data]
  Gateway Out7/1 -> rd_wr_debug/3
  Gateway Out5/1 -> rd_wr_debug/2
  Gateway Out6/1 -> rd_wr_debug/1
  Slice2/1 -> RB_done/1
  fifo_out/1 -> Slice5/1, Slice2/1, Slice1/1
  Convert1/1 -> Concat1/1
  [rb_done] -> Convert1/1
  Concat1/1 -> fifo_out/1
  [qdr_data] -> Concat1/2
  [rb_en] -> fifo_out/2
  ack_RB/1 -> [out_ack], fifo_out/3
  [out_ack] -> Logical6/1
  Slice15/1 -> delay4/1
  [in_burst_rdy] -> acc_ctrl/1(input_burst_rdy)
  fifo_in/1 -> Gateway Out4/1, delay2/1
  acc_ctrl/4(fifo_rd_en) -> [fifo_rd_en]
  Constant3/1 -> qdr/3
  qdr/1 -> make_odd_delay/1
  acc_ctrl/3(address) -> Gateway Out7/1, qdr/4, [qdr_addr]
  acc_ctrl/2(wr_en) -> Gateway Out5/1, qdr/2, [qdr_wr_en]
  acc_ctrl/1(rd_en) -> Gateway Out6/1, qdr/1, [qdr_rd_en]
  Concat/1 -> delay/1
  valid_data/1 -> Logical2/1, Gateway Out3/1, [valid_in]
  data_in/1 -> Assert/1
  fifo_in/3 -> Slice15/1
  [cal_fail] -> Concat2/5, Logical1/1
  [input_overflow] -> Concat2/4, Logical1/2
  [rst] -> Concat2/3, Logical1/3
  [output_over] -> Logical1/4, Concat2/2
  Slice1/1 -> data_out/1
  Gateway Out31/1 -> input_debug/4
  [rst] -> Gateway Out31/1
  [rst] -> rst_delay/1
  Inverter1/1 -> Logical6/2
  fifo_out/2 -> Inverter1/1
  Logical6/1 -> out_valid_delay/1
  qdr_del_comp2/1 -> Gateway Out15/1
  qdr_del_comp3/1 -> Gateway Out14/1
  qdr_del_comp4/1 -> Gateway Out28/1
  qdr_del_comp5/1 -> Gateway Out11/1
  qdr_del_comp6/1 -> Gateway Out19/1
  qdr_del_comp7/1 -> Gateway Out22/1
  [fifo_rd_en] -> fifo_in/3
  rst_delay/1 -> fifo_out/4
  fifo_in/2 -> Terminator1/1
  delay/1 -> fifo_in/1
  delay1/1 -> fifo_in/2
  acc_ctrl/8(new_acc) -> [new_acc]
  [new_acc] -> stat_del15/1
  stat_del15/1 -> new_acc (ASYNC)/1
  [new_acc] -> qdr_del_comp8/1
  Gateway Out33/1 -> acc_debug/10
  qdr_del_comp8/1 -> Gateway Out33/1
  out_valid_delay/1 -> valid/1
  Inverter2/1 -> Logical2/3
  [rst] -> Inverter2/1
  Slice3/1 -> [output_full], pkt_rdy/1
  Constant/1 -> Relational/2
  Relational/1 -> Logical4/2, Gateway Out38/1
  sync_count/1 -> Gateway Out24/1, Relational/1
  Gateway Out30/1 -> sync_debug/3
  Gateway Out24/1 -> sync_debug/2
  Gateway Out29/1 -> sync_debug/1
  [valid_in] -> sync_count/2
  Gateway Out32/1 -> sync_debug/4
  [unbuf_in_data] -> Gateway Out32/1
  Logical7/1 -> delay5/1
  Gateway Out36/1 -> sync_debug/5
  [valid_in] -> Gateway Out36/1
  Gateway Out37/1 -> sync_debug/6
  Gateway Out38/1 -> sync_debug/7
  sync/1 -> Logical5/2, Gateway Out29/1, Gateway Out43/1, Logical3/1
  [valid_in] -> Logical4/1
  Logical5/1 -> sync_count/1, Gateway Out37/1
  Inverter/1 -> Gateway Out50/1, Logical3/2
  Logical4/1 -> Register/3, Logical8/1, Register/1, Logical5/3
  Logical3/1 -> Gateway Out51/1, Logical7/2
  [rst] -> Gateway Out30/1
  rst/1 -> Logical7/1, Gateway Out39/1, Logical5/1
  Logical8/1 -> Inverter/1
  Register/1 -> Gateway Out49/1, Logical9/2, Logical10/1
  [valid_in] -> Logical9/1
  Logical9/1 -> Register/2
  Inverter3/1 -> Logical10/2
  Logical10/1 -> Logical8/2
  [valid_in] -> Inverter3/1
  delay3/1 -> Logical11/2
  Logical11/1 -> fifo_in/4
  [rst] -> delay3/1, Logical11/1
  Convert/1 -> parity_insertion/1(din)
  parity_insertion/1(dout) -> qdr/5
  [parity_error] -> Concat2/1, Logical1/5
  Slice4/1 -> [qdr_data]
  [qdr_valid] -> Gateway Out35/1
  [qdr_data] -> Slice7/1
  bus_expand/2(lsb_out1) -> Gateway Out41/1
  [qdr_wr_en] -> Gateway Out42/1
  [acc_data] -> Slice6/1
  bus_expand1/2(lsb_out1) -> Gateway Out45/1
  bus_expand1/1(msb_out2) -> Gateway Out44/1
  [qdr_rd_en] -> Gateway Out46/1
  [qdr_addr] -> Gateway Out47/1
  Slice6/1 -> bus_expand1/1(bus_in)
  Slice7/1 -> bus_expand/1(bus_in)
  bus_expand/1(msb_out2) -> Gateway Out40/1
  Gateway Out45/1 -> qdr_in/5
  Gateway Out47/1 -> qdr_in/3
  Gateway Out42/1 -> qdr_in/1
  Gateway Out35/1 -> qdr_in/6
  Gateway Out44/1 -> qdr_in/4
  Gateway Out46/1 -> qdr_in/2
  Gateway Out40/1 -> qdr_in/7
  Gateway Out41/1 -> qdr_in/8
  Gateway Out39/1 -> rst_debug/1
  Gateway Out43/1 -> rst_debug/2
  [valid_in] -> Gateway Out48/1
  Gateway Out48/1 -> rst_debug/3
  Gateway Out49/1 -> rst_debug/4
  Gateway Out50/1 -> rst_debug/5
  Gateway Out51/1 -> rst_debug/6
  Gateway Out52/1 -> rst_debug/7
  parity_check/1(error) -> [parity_error]
  Concat2/1 -> error_flags/1

== system r2_b16a4x512f/sys0/vacc/rst_replicate ==
  in : Inport
  bussify : Subsystem  AncestorBlock=casper_library_flow_control/bus_create  mask(bus_create){inputNum=19}
      mask prompts: inputNum "Number of inputs:"
      mask init:
      | bus_create_init(gcb,...
      |     'inputNum', inputNum);
  out : Outport
  wires:
  in/1 -> bussify/1(in1), bussify/2(in2), bussify/3(in3), bussify/4(in4), bussify/5(in5), bussify/6(in6), bussify/7(in7), bussify/8(in8), bussify/9(in9), bussify/10(in10), bussify/11(in11), bussify/12(in12), bussify/13(in13), bussify/14(in14), bussify/15(in15), bussify/16(in16), bussify/17(in17), bussify/18(in18), bussify/19(in19)
  bussify/1(bus_out) -> out/1

== system r2_b16a4x512f/sys0/vacc/vacc_rst ==
  rst : Inport
  arm : Inport  Port=2
  load_time : Inport  Port=3
  current_time : Inport  Port=4
  immediate : Inport  Port=5
  Delay : xbsIndex_r4/Delay  rst=off  infoeditControl=Selection of Reset will increase slice count due to use of real FFs and instead of SRLs  en=off  latency=1  dbl_ovrd=off  reg_retiming=on  block_type=delay
  Gateway Out{,1..3} (4 alike) : xbsIndex_r4/Gateway Out  inherit_from_input=off  hdl_port=on  timing_constraint=None  locs_specified=off  LOCs={}  UseAsDAC=off  DACChannel='1'  block_type=gatewayout
  Logical : xbsIndex_r4/Logical  logical_function=OR  inputs=2  en=off  latency=0  precision=Full  arith_type=Unsigned  n_bits=16  bin_pt=0  align_bp=on  dbl_ovrd=off  block_type=logical
  Logical1 : xbsIndex_r4/Logical  logical_function=AND  inputs=2  en=off  latency=0  precision=Full  arith_type=Unsigned  n_bits=16  bin_pt=0  align_bp=on  dbl_ovrd=off  block_type=logical
  Logical2 : xbsIndex_r4/Logical  logical_function=OR  inputs=2  en=off  latency=0  precision=Full  arith_type=Unsigned  n_bits=16  bin_pt=0  align_bp=on  dbl_ovrd=off  block_type=logical
  Register2 : xbsIndex_r4/Register  init=0  rst=off  en=on  dbl_ovrd=off  block_type=register
  Register3 : xbsIndex_r4/Register  init=0  rst=on  en=on  dbl_ovrd=off  block_type=register
  Relational : xbsIndex_r4/Relational  mode=a=b  en=off  latency=1  dbl_ovrd=off  block_type=relational
      settings: block_version=10.1.3
  Scope : Scope  NumInputPorts=4
      settings: YMin=-5~-5~-5~-5  YMax=5~5~5~5  SaveName=ScopeData11
  armed : xbsIndex_r4/Register  init=0  rst=on  en=on  dbl_ovrd=off  block_type=register
  count0 : xbsIndex_r4/Counter  cnt_type=Free Running  cnt_to=Inf  operation=Up  start_count=0  cnt_by_val=1  arith_type=Unsigned  n_bits=cnt_bits  bin_pt=0  load_pin=off  rst=on  en=on  explicit_period=on  period=1  dbl_ovrd=off  use_behavioral_HDL=off  implementation=Fabric  block_type=counter
      settings: block_version=11.4
  count1 : xbsIndex_r4/Counter  cnt_type=Free Running  cnt_to=Inf  operation=Up  start_count=0  cnt_by_val=1  arith_type=Unsigned  n_bits=cnt_bits  bin_pt=0  load_pin=off  rst=on  en=on  explicit_period=on  period=1  dbl_ovrd=off  use_behavioral_HDL=off  implementation=Fabric  block_type=counter
      settings: block_version=11.4
  edge_detect : Subsystem  AncestorBlock=casper_library_misc/edge_detect  mask(edge_detect){edge=Rising, polarity=Active High, x_in=[0 0.08 0.08 0.16 0.16 0.24 0.24 0.32 0.32 0.4], y_in=[-1 -1  1  1  1  1  1  1  1  1], x_out=[0.6 0.68 0.68 0.76 0.76 0.84 0.84 0.92 0.92 1], y_out=[-1 -1  1  1 -1 -1 -1 -1 -1 -1]}
      mask prompts: edge "Edge Type"; polarity "Output Polarity"; x_in "Input X Positions"; y_in "Input Y Positions"; x_out "Output X Positions"; y_out "Output Y Positions"
      mask help: Output is active for one-cycle after each edge of the specified type (i.e. rising, falling or both).
      mask init: same as r2_b16a4x512f/edge_detect
      settings: AttributesFormatString=|
      | rising edges
      | active high
      mask Help: Output is active for one-cycle after each edge of the specified type (i.e. rising, falling, or both).  Latency is zero.
      mask TypeOptions edge: Rising | Falling | Both
      mask TypeOptions polarity: Active High | Active Low
      mask Display:
      | plot(x_in_num,0.5+y_in_num*0.2);
      | plot(x_out_num,0.5+y_out_num*0.2);
  edge_detect1 : Subsystem  AncestorBlock=casper_library_misc/edge_detect  mask(edge_detect){edge=Rising, polarity=Active High, x_in=[0 0.08 0.08 0.16 0.16 0.24 0.24 0.32 0.32 0.4], y_in=[-1 -1  1  1  1  1  1  1  1  1], x_out=[0.6 0.68 0.68 0.76 0.76 0.84 0.84 0.92 0.92 1], y_out=[-1 -1  1  1 -1 -1 -1 -1 -1 -1]}
      mask prompts: edge "Edge Type"; polarity "Output Polarity"; x_in "Input X Positions"; y_in "Input Y Positions"; x_out "Output X Positions"; y_out "Output Y Positions"
      mask help: Output is active for one-cycle after each edge of the specified type (i.e. rising, falling or both).
      mask init: same as r2_b16a4x512f/edge_detect
      settings: AttributesFormatString=|
      | rising edges
      | active high
      mask Help: Output is active for one-cycle after each edge of the specified type (i.e. rising, falling, or both).  Latency is zero.
      mask TypeOptions edge: Rising | Falling | Both
      mask TypeOptions polarity: Active High | Active Low
      mask Display:
      | plot(x_in_num,0.5+y_in_num*0.2);
      | plot(x_out_num,0.5+y_out_num*0.2);
  edge_detect2 : Subsystem  AncestorBlock=casper_library_misc/edge_detect  mask(edge_detect){edge=Rising, polarity=Active High, x_in=[0 0.08 0.08 0.16 0.16 0.24 0.24 0.32 0.32 0.4], y_in=[-1 -1  1  1  1  1  1  1  1  1], x_out=[0.6 0.68 0.68 0.76 0.76 0.84 0.84 0.92 0.92 1], y_out=[-1 -1  1  1 -1 -1 -1 -1 -1 -1]}
      mask prompts: edge "Edge Type"; polarity "Output Polarity"; x_in "Input X Positions"; y_in "Input Y Positions"; x_out "Output X Positions"; y_out "Output Y Positions"
      mask help: Output is active for one-cycle after each edge of the specified type (i.e. rising, falling or both).
      mask init: same as r2_b16a4x512f/edge_detect
      settings: AttributesFormatString=|
      | rising edges
      | active high
      mask Help: Output is active for one-cycle after each edge of the specified type (i.e. rising, falling, or both).  Latency is zero.
      mask TypeOptions edge: Rising | Falling | Both
      mask TypeOptions polarity: Active High | Active Low
      mask Display:
      | plot(x_in_num,0.5+y_in_num*0.2);
      | plot(x_out_num,0.5+y_out_num*0.2);
  edge_detect3 : Subsystem  AncestorBlock=casper_library_misc/edge_detect  mask(edge_detect){edge=Rising, polarity=Active High, x_in=[0 0.08 0.08 0.16 0.16 0.24 0.24 0.32 0.32 0.4], y_in=[-1 -1  1  1  1  1  1  1  1  1], x_out=[0.6 0.68 0.68 0.76 0.76 0.84 0.84 0.92 0.92 1], y_out=[-1 -1  1  1 -1 -1 -1 -1 -1 -1]}
      mask prompts: edge "Edge Type"; polarity "Output Polarity"; x_in "Input X Positions"; y_in "Input Y Positions"; x_out "Output X Positions"; y_out "Output Y Positions"
      mask help: Output is active for one-cycle after each edge of the specified type (i.e. rising, falling or both).
      mask init: same as r2_b16a4x512f/edge_detect
      settings: AttributesFormatString=|
      | rising edges
      | active high
      mask Help: Output is active for one-cycle after each edge of the specified type (i.e. rising, falling, or both).  Latency is zero.
      mask TypeOptions edge: Rising | Falling | Both
      mask TypeOptions polarity: Active High | Active Low
      mask Display:
      | plot(x_in_num,0.5+y_in_num*0.2);
      | plot(x_out_num,0.5+y_out_num*0.2);
  arm_count : Outport
  ld_count : Outport  Port=2
  enable : Outport  Port=3
  wires:
  edge_detect1/1(out) -> Gateway Out/1, Register3/2, armed/3, armed/1
  Logical2/1 -> armed/2
  edge_detect/1(out) -> count0/2
  current_time/1 -> Relational/1
  arm/1 -> edge_detect1/1(in), Register2/2
  Logical1/1 -> Register3/3, Register3/1, count1/2
  armed/1 -> edge_detect/1(in), Gateway Out1/1, Logical1/1
  Register3/1 -> Gateway Out3/1, enable/1
  rst/1 -> count1/1, count0/1, Logical2/1
  count0/1 -> arm_count/1
  count1/1 -> ld_count/1
  load_time/1 -> Register2/1
  Register2/1 -> Relational/2
  immediate/1 -> Delay/1
  Relational/1 -> edge_detect2/1(in)
  Delay/1 -> edge_detect3/1(in)
  Gateway Out/1 -> Scope/1
  Gateway Out1/1 -> Scope/2
  Gateway Out2/1 -> Scope/3
  Gateway Out3/1 -> Scope/4
  edge_detect2/1(out) -> Logical/1
  edge_detect3/1(out) -> Logical/2
  Logical/1 -> Gateway Out2/1, Logical1/2, Logical2/2

== system r2_b16a4x512f/sys0/vacc/zeros ==
  bus_create : Subsystem  AncestorBlock=casper_library_flow_control/bus_create  mask(bus_create){inputNum=19}
      mask prompts: inputNum "Number of inputs:"
      mask init:
      | bus_create_init(gcb,...
      |     'inputNum', inputNum);
  constant{0..18} (19 alike) : xbsIndex_r4/Constant  const=0  gui_display_data_type=Fixed-point  arith_type=Unsigned  n_bits=1  bin_pt=0  preci_type=Single  exp_width=8  frac_width=24  explicit_period=on  period=1  equ=P=C  opselect=C  inp2=PCIN>>17  opr=+  inp1=P  carry=CIN  dbl_ovrd=off  block_type=constant
  dout : Outport
  wires:
  constant0/1 -> bus_create/1(in1)
  constant1/1 -> bus_create/2(in2)
  constant2/1 -> bus_create/3(in3)
  constant3/1 -> bus_create/4(in4)
  constant4/1 -> bus_create/5(in5)
  constant5/1 -> bus_create/6(in6)
  constant6/1 -> bus_create/7(in7)
  constant7/1 -> bus_create/8(in8)
  constant8/1 -> bus_create/9(in9)
  constant9/1 -> bus_create/10(in10)
  constant10/1 -> bus_create/11(in11)
  constant11/1 -> bus_create/12(in12)
  constant12/1 -> bus_create/13(in13)
  constant13/1 -> bus_create/14(in14)
  constant14/1 -> bus_create/15(in15)
  constant15/1 -> bus_create/16(in16)
  constant16/1 -> bus_create/17(in17)
  constant17/1 -> bus_create/18(in18)
  constant18/1 -> bus_create/19(in19)
  bus_create/1(bus_out) -> dout/1

== system r2_b16a4x512f/sys0/vacc_tvg0/bus_replicate ==
  in : Inport
  bussify : Subsystem  AncestorBlock=casper_library_flow_control/bus_create  mask(bus_create){inputNum=2}
      mask prompts: inputNum "Number of inputs:"
      mask init:
      | bus_create_init(gcb,...
      |     'inputNum', inputNum);
  out : Outport
  wires:
  in/1 -> bussify/1(in1), bussify/2(in2)
  bussify/1(bus_out) -> out/1

== system r2_b16a4x512f/sys0/vacc_tvg0/bus_replicate1 ==
  in : Inport
  bussify : Subsystem  AncestorBlock=casper_library_flow_control/bus_create  mask(bus_create){inputNum=2}
      mask prompts: inputNum "Number of inputs:"
      mask init:
      | bus_create_init(gcb,...
      |     'inputNum', inputNum);
  out : Outport
  wires:
  bussify/1(bus_out) -> out/1
  in/1 -> bussify/2(in2), bussify/1(in1)

== system r2_b16a4x512f/sys0/vacc_tvg0/edge_detect ==
  in : Inport
  Delay : xbsIndex_r4/Delay  rst=off  infoeditControl=Selection of Reset will increase slice count due to use of real FFs and instead of SRLs  en=off  latency=1  dbl_ovrd=off  reg_retiming=on  block_type=delay
      settings: xl_area=[0, 0, 0, 0, 0, 0, 0]
  Inverter : xbsIndex_r4/Inverter  en=off  latency=0  dbl_ovrd=off  block_type=inv
      settings: xl_area=[0, 0, 0, 0, 0, 0, 0]
  edge_op : xbsIndex_r4/Logical  logical_function=NOR  inputs=2  en=off  latency=0  precision=Full  arith_type=Unsigned  n_bits=8  bin_pt=2  align_bp=on  dbl_ovrd=off  block_type=logical
      settings: xl_area=[0, 0, 0, 0, 0, 0, 0]
  out : Outport
  wires:
  Delay/1 -> edge_op/2
  in/1 -> Delay/1, Inverter/1
  edge_op/1 -> out/1
  Inverter/1 -> edge_op/1
